simulink model "IEEE9BusSystem"  (R2024a)
settings: Solver=FixedStepAuto  StartTime=0  StopTime=100  FixedStep=Ts  RelTol=1e-3  AbsTol=1e-3  EnableMultiTasking=on
PreLoadFcn:
  | Ts = 1/60;
libraries: ee_lib x63, nesl_utility x48, fl_lib x22, eeGeneralControl x6, spsFrequencyPhasorLib x3, eeSmAC1C x3, eeSmPSS1A x3, spspowerguiLib x1
(part 2 of 2)

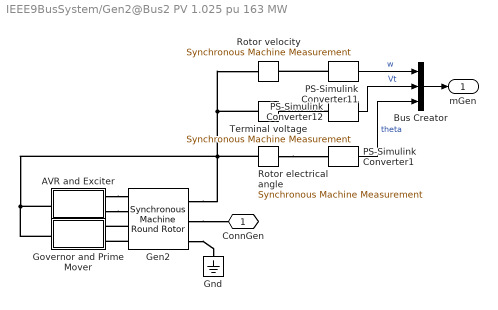
== system IEEE9BusSystem/Gen2@Bus2 PV 1.025 pu 163 MW ==
  AVR and Exciter : Subsystem
  Bus Creator : BusCreator  Inputs=3
  Gen2 : ee_lib/Electromechanical/Synchronous/Synchronous Machine Round Rotor  port_option=ee.enum.threePhasePort.composite  SRated=192 MW  VRated=18 kV  FRated=60 Hz  nPolePairs=1  param_option=ee.enum.sm.parameterization.standard  fieldCircuitParameterization_option=ee.enum.sm.fieldparameterization.current  baseEfd=92.95 V  baseIfd=100 A  zero_sequence=ee.enum.park.zerosequence.include  axes_param=ee.enum.rotorangle.qaxis  Ladu=1.6801  Laqu=1.62  L0=0.0399  Ll=0.0399  Ra=0.01  Lfd=0.2162  Rfd=8.558e-4  L1d=0.4343  R1d=0.0325  L1q=0.2635  R1q=0.0326  L2q=0.4627  R2q=0.0131  Xl=0.1  Xd=1.7199  Xq=1.6598  X0=0.1  Xdd=0.23  Xqd=0.378  Xddd=0.1728  Xqdd=0.192  d_option=ee.enum.circuit.open  Td0d=6 s  Tdd=1.3260 s  Td0dd=0.05 s  Tddd=0.0230 s  q_option=ee.enum.circuit.open  Tq0d=0.535 s  Tqd=0.3693 s  Tq0dd=0.04 s  Tqdd=0.0269 s  saturation_option=ee.enum.saturation.exclude  saturation_ifd=[0.0, 0.48, 0.76, 1.38, 1.79]  saturation_Vag=[0.0, 0.8, 1.08, 1.31, 1.4]  initialization_option=ee.enum.sm.initialization.steadystate  source_type=ee.enum.sm.load_flow_source_type.PV  Vmag0=18*1.025 kV  Vang0=0 deg  Pt0=163 MW  Qt0=0 V*A  minimum_pu=0.95  phase_search_range=[-30, 30] deg  gmin=1e-6 S  connection_option=ee.enum.Connection.wye  num_q_dampers=2  rotor_offset=-pi / 2 rad  pu_psid_specify=on  pu_psid_priority=High  pu_psid=0  pu_psid_nominal_specify=off  pu_psid_nominal_value=1  pu_psid_nominal_unit=1  pu_psiq_specify=on  pu_psiq_priority=High  pu_psiq=0  pu_psiq_nominal_specify=off  pu_psiq_nominal_value=1  pu_psiq_nominal_unit=1  pu_psifd_specify=on  pu_psifd_priority=High  pu_psifd=0  pu_psifd_nominal_specify=off  pu_psifd_nominal_value=1  pu_psifd_nominal_unit=1  pu_psi1d_specify=on  pu_psi1d_priority=High  pu_psi1d=0  pu_psi1d_nominal_specify=off  pu_psi1d_nominal_value=1  pu_psi1d_nominal_unit=1  pu_psi1q_specify=on  pu_psi1q_priority=High  pu_psi1q=0  pu_psi1q_nominal_specify=off  pu_psi1q_nominal_value=1  pu_psi1q_nominal_unit=1  pu_psi2q_specify=on  pu_psi2q_priority=High  pu_psi2q=0  pu_psi2q_nominal_specify=off  pu_psi2q_nominal_value=1  pu_psi2q_nominal_unit=1  angular_position_diff_specify=off  angular_position_diff_priority=None  angular_position_diff=0 deg  angular_position_diff_nominal_specify=off  angular_position_diff_nominal_value=1  angular_position_diff_nominal_unit=deg  Tmeas=298.15 K  alpha=3.93e-3 1/K  stator_thermal_mass=100 J/K  rotor_thermal_mass=200 J/K  temperatureA_specify=off  temperatureA_priority=High  temperatureA=25 degC  temperatureA_nominal_specify=off  temperatureA_nominal_value=1  temperatureA_nominal_unit=degC  temperatureB_specify=off  temperatureB_priority=High  temperatureB=25 degC  temperatureB_nominal_specify=off  temperatureB_nominal_value=1  temperatureB_nominal_unit=degC  temperatureC_specify=off  temperatureC_priority=High  temperatureC=25 degC  temperatureC_nominal_specify=off  temperatureC_nominal_value=1  temperatureC_nominal_unit=degC  temperatureR_specify=off  temperatureR_priority=High  temperatureR=25 degC  temperatureR_nominal_specify=off  temperatureR_nominal_value=1  temperatureR_nominal_unit=degC
      settings: InternalSimscapePortConfiguration="{\"Bottom\":[],\"Left\":[{\"id\":\"fd_p\",\"label\":\"fd+\",\"type\":\"foundation.electrical.electrical\"},{\"id\":\"fd_n\",\"label\":\"fd-\",\"type\":\"foundation.electrical.electrical\"},{\"id\":\"R\",\"label\":\"R\",\"type\":\"foundation.mechanical.rotational.rotational\"},{\"id\":\"C\",\"label\":\"C\",\"type\":\"foundation.mechanical.rotational.rotational\"}],\"Right\":[{\"id\":\"pu_output\",\"label\":\"pu\",\"type\":\"output\"},{\"id\":\"N\",\"label\":\"~\",\"type\":\"foundation.electrical.three_phase\"},{\"id\":\"n\",\"label\":\"n\",\"type\":\"foundation.electrical.electrical\"}],\"Top\":[]}"
  Gnd : fl_lib/Electrical/Electrical Elements/Electrical Reference
  Governor and Prime Mover : Subsystem
  PS-Simulink Converter1 : nesl_utility/PS-Simulink Converter  PhysicalDomain=network_engine_domain  SubClassName=ps_output  LeftPortType=input  RightPortType=output  PseudoPeriodic=off  Frequencies=[]  VectorFormat=1-D array  Unit=1  AffineConversion=off
  PS-Simulink Converter11 : nesl_utility/PS-Simulink Converter  PhysicalDomain=network_engine_domain  SubClassName=ps_output  LeftPortType=input  RightPortType=output  PseudoPeriodic=off  Frequencies=[]  VectorFormat=1-D array  Unit=1  AffineConversion=off
  PS-Simulink Converter12 : nesl_utility/PS-Simulink Converter  PhysicalDomain=network_engine_domain  SubClassName=ps_output  LeftPortType=input  RightPortType=output  PseudoPeriodic=off  Frequencies=[]  VectorFormat=1-D array  Unit=1  AffineConversion=off
  Rotor electrical angle : ee_lib/Electromechanical/Synchronous/Synchronous Machine Measurement  output_idx=19
      settings: InternalSimscapePortConfiguration="{\"Bottom\":[],\"Left\":[{\"id\":\"pu_input\",\"label\":\"pu\",\"type\":\"input\"}],\"Right\":[{\"id\":\"pu_output\",\"label\":\"o\",\"type\":\"output\"}],\"Top\":[]}"
  Rotor velocity : ee_lib/Electromechanical/Synchronous/Synchronous Machine Measurement  output_idx=4
      settings: InternalSimscapePortConfiguration="{\"Bottom\":[],\"Left\":[{\"id\":\"pu_input\",\"label\":\"pu\",\"type\":\"input\"}],\"Right\":[{\"id\":\"pu_output\",\"label\":\"o\",\"type\":\"output\"}],\"Top\":[]}"
  Terminal voltage : ee_lib/Electromechanical/Synchronous/Synchronous Machine Measurement  output_idx=14
      settings: InternalSimscapePortConfiguration="{\"Bottom\":[],\"Left\":[{\"id\":\"pu_input\",\"label\":\"pu\",\"type\":\"input\"}],\"Right\":[{\"id\":\"pu_output\",\"label\":\"o\",\"type\":\"output\"}],\"Top\":[]}"
  ConnGen : PMIOPort  Side=Right
  mGen : Outport
  wires:
  PS-Simulink Converter11/1 -> Bus Creator/1  "w"
  Bus Creator/1 -> mGen/1
  PS-Simulink Converter12/1 -> Bus Creator/2  "Vt"
  PS-Simulink Converter1/1 -> Bus Creator/3  "theta"
  connections:
  AVR and Exciter/RConn1 -- Gen2/LConn1
  AVR and Exciter/RConn2 -- Gen2/LConn2
  Gen2/LConn3 -- Governor and Prime Mover/RConn1
  Gen2/LConn4 -- Governor and Prime Mover/RConn2
  Gen2/RConn2 -- ConnGen/RConn1
  Gen2/RConn3 -- Gnd/LConn1
  Gen2/RConn1 -- AVR and Exciter/LConn1 -- Governor and Prime Mover/LConn1 -- Rotor electrical angle/LConn1 -- Rotor velocity/LConn1 -- Terminal voltage/LConn1
  PS-Simulink Converter11/LConn1 -- Rotor velocity/RConn1
  PS-Simulink Converter12/LConn1 -- Terminal voltage/RConn1
  Rotor electrical angle/RConn1 -- PS-Simulink Converter1/LConn1

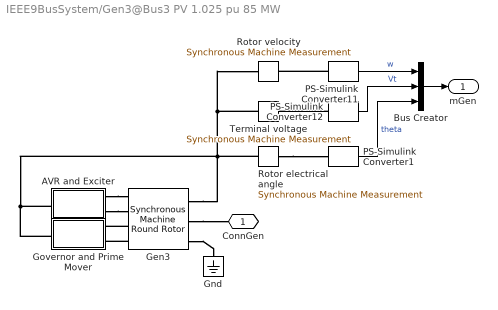
== system IEEE9BusSystem/Gen3@Bus3 PV 1.025 pu 85 MW ==
  AVR and Exciter : Subsystem
  Bus Creator : BusCreator  Inputs=3
  Gen3 : ee_lib/Electromechanical/Synchronous/Synchronous Machine Round Rotor  port_option=ee.enum.threePhasePort.composite  SRated=128 MW  VRated=13.8 kV  FRated=60 Hz  nPolePairs=1  param_option=ee.enum.sm.parameterization.standard  fieldCircuitParameterization_option=ee.enum.sm.fieldparameterization.current  baseEfd=92.95 V  baseIfd=100 A  zero_sequence=ee.enum.park.zerosequence.include  axes_param=ee.enum.rotorangle.qaxis  Ladu=1.5958  Laqu=1.5257  L0=0.0842  Ll=0.0842  Ra=0.01  Lfd=0.1715  Rfd=8.4749e-4  L1d=0.061  R1d=0.0108  L1q=0.1726  R1q=0.0222  L2q=0.3535  R2q=0.0144  Xl=0.095  Xd=1.68  Xq=1.61  X0=0.095  Xdd=0.2321  Xqd=0.32  Xddd=0.128  Xqdd=0.192  d_option=ee.enum.circuit.open  Td0d=5.89 s  Tdd=1.3260 s  Td0dd=0.05 s  Tddd=0.0230 s  q_option=ee.enum.circuit.open  Tq0d=0.6 s  Tqd=0.3693 s  Tq0dd=0.04 s  Tqdd=0.0269 s  saturation_option=ee.enum.saturation.exclude  saturation_ifd=[0.0, 0.48, 0.76, 1.38, 1.79]  saturation_Vag=[0.0, 0.8, 1.08, 1.31, 1.4]  initialization_option=ee.enum.sm.initialization.steadystate  source_type=ee.enum.sm.load_flow_source_type.PV  Vmag0=13.8*1.025 kV  Vang0=0 deg  Pt0=85 MW  Qt0=0 V*A  minimum_pu=0.95  phase_search_range=[-30, 30] deg  gmin=1e-6 S  connection_option=ee.enum.Connection.wye  num_q_dampers=2  rotor_offset=-pi / 2 rad  pu_psid_specify=on  pu_psid_priority=High  pu_psid=0  pu_psid_nominal_specify=off  pu_psid_nominal_value=1  pu_psid_nominal_unit=1  pu_psiq_specify=on  pu_psiq_priority=High  pu_psiq=0  pu_psiq_nominal_specify=off  pu_psiq_nominal_value=1  pu_psiq_nominal_unit=1  pu_psifd_specify=on  pu_psifd_priority=High  pu_psifd=0  pu_psifd_nominal_specify=off  pu_psifd_nominal_value=1  pu_psifd_nominal_unit=1  pu_psi1d_specify=on  pu_psi1d_priority=High  pu_psi1d=0  pu_psi1d_nominal_specify=off  pu_psi1d_nominal_value=1  pu_psi1d_nominal_unit=1  pu_psi1q_specify=on  pu_psi1q_priority=High  pu_psi1q=0  pu_psi1q_nominal_specify=off  pu_psi1q_nominal_value=1  pu_psi1q_nominal_unit=1  pu_psi2q_specify=on  pu_psi2q_priority=High  pu_psi2q=0  pu_psi2q_nominal_specify=off  pu_psi2q_nominal_value=1  pu_psi2q_nominal_unit=1  angular_position_diff_specify=off  angular_position_diff_priority=High  angular_position_diff=0 deg  angular_position_diff_nominal_specify=off  angular_position_diff_nominal_value=1  angular_position_diff_nominal_unit=deg  Tmeas=298.15 K  alpha=3.93e-3 1/K  stator_thermal_mass=100 J/K  rotor_thermal_mass=200 J/K  temperatureA_specify=off  temperatureA_priority=High  temperatureA=25 degC  temperatureA_nominal_specify=off  temperatureA_nominal_value=1  temperatureA_nominal_unit=degC  temperatureB_specify=off  temperatureB_priority=High  temperatureB=25 degC  temperatureB_nominal_specify=off  temperatureB_nominal_value=1  temperatureB_nominal_unit=degC  temperatureC_specify=off  temperatureC_priority=High  temperatureC=25 degC  temperatureC_nominal_specify=off  temperatureC_nominal_value=1  temperatureC_nominal_unit=degC  temperatureR_specify=off  temperatureR_priority=High  temperatureR=25 degC  temperatureR_nominal_specify=off  temperatureR_nominal_value=1  temperatureR_nominal_unit=degC
      settings: InternalSimscapePortConfiguration="{\"Bottom\":[],\"Left\":[{\"id\":\"fd_p\",\"label\":\"fd+\",\"type\":\"foundation.electrical.electrical\"},{\"id\":\"fd_n\",\"label\":\"fd-\",\"type\":\"foundation.electrical.electrical\"},{\"id\":\"R\",\"label\":\"R\",\"type\":\"foundation.mechanical.rotational.rotational\"},{\"id\":\"C\",\"label\":\"C\",\"type\":\"foundation.mechanical.rotational.rotational\"}],\"Right\":[{\"id\":\"pu_output\",\"label\":\"pu\",\"type\":\"output\"},{\"id\":\"N\",\"label\":\"~\",\"type\":\"foundation.electrical.three_phase\"},{\"id\":\"n\",\"label\":\"n\",\"type\":\"foundation.electrical.electrical\"}],\"Top\":[]}"
  Gnd : fl_lib/Electrical/Electrical Elements/Electrical Reference
  Governor and Prime Mover : Subsystem
  PS-Simulink Converter1 : nesl_utility/PS-Simulink Converter  PhysicalDomain=network_engine_domain  SubClassName=ps_output  LeftPortType=input  RightPortType=output  PseudoPeriodic=off  Frequencies=[]  VectorFormat=1-D array  Unit=1  AffineConversion=off
  PS-Simulink Converter11 : nesl_utility/PS-Simulink Converter  PhysicalDomain=network_engine_domain  SubClassName=ps_output  LeftPortType=input  RightPortType=output  PseudoPeriodic=off  Frequencies=[]  VectorFormat=1-D array  Unit=1  AffineConversion=off
  PS-Simulink Converter12 : nesl_utility/PS-Simulink Converter  PhysicalDomain=network_engine_domain  SubClassName=ps_output  LeftPortType=input  RightPortType=output  PseudoPeriodic=off  Frequencies=[]  VectorFormat=1-D array  Unit=1  AffineConversion=off
  Rotor electrical angle : ee_lib/Electromechanical/Synchronous/Synchronous Machine Measurement  output_idx=19
      settings: InternalSimscapePortConfiguration="{\"Bottom\":[],\"Left\":[{\"id\":\"pu_input\",\"label\":\"pu\",\"type\":\"input\"}],\"Right\":[{\"id\":\"pu_output\",\"label\":\"o\",\"type\":\"output\"}],\"Top\":[]}"
  Rotor velocity : ee_lib/Electromechanical/Synchronous/Synchronous Machine Measurement  output_idx=4
      settings: InternalSimscapePortConfiguration="{\"Bottom\":[],\"Left\":[{\"id\":\"pu_input\",\"label\":\"pu\",\"type\":\"input\"}],\"Right\":[{\"id\":\"pu_output\",\"label\":\"o\",\"type\":\"output\"}],\"Top\":[]}"
  Terminal voltage : ee_lib/Electromechanical/Synchronous/Synchronous Machine Measurement  output_idx=14
      settings: InternalSimscapePortConfiguration="{\"Bottom\":[],\"Left\":[{\"id\":\"pu_input\",\"label\":\"pu\",\"type\":\"input\"}],\"Right\":[{\"id\":\"pu_output\",\"label\":\"o\",\"type\":\"output\"}],\"Top\":[]}"
  ConnGen : PMIOPort  Side=Right
  mGen : Outport
  wires:
  PS-Simulink Converter1/1 -> Bus Creator/3  "theta"
  PS-Simulink Converter12/1 -> Bus Creator/2  "Vt"
  Bus Creator/1 -> mGen/1
  PS-Simulink Converter11/1 -> Bus Creator/1  "w"
  connections:
  Rotor electrical angle/RConn1 -- PS-Simulink Converter1/LConn1
  PS-Simulink Converter12/LConn1 -- Terminal voltage/RConn1
  PS-Simulink Converter11/LConn1 -- Rotor velocity/RConn1
  Terminal voltage/LConn1 -- Gen3/RConn1 -- Rotor electrical angle/LConn1 -- AVR and Exciter/LConn1 -- Governor and Prime Mover/LConn1 -- Rotor velocity/LConn1
  Gen3/RConn3 -- Gnd/LConn1
  Gen3/RConn2 -- ConnGen/RConn1
  Gen3/LConn4 -- Governor and Prime Mover/RConn2
  Gen3/LConn3 -- Governor and Prime Mover/RConn1
  AVR and Exciter/RConn2 -- Gen3/LConn2
  AVR and Exciter/RConn1 -- Gen3/LConn1

== system IEEE9BusSystem/Scope ==
  BusElementIn : Inport  PortName=mGen1  Element=w
  BusElementIn1 : Inport  PortName=mGen1  Element=Vt
  BusElementIn2 : Inport  Port=2  PortName=mGen2  Element=Vt
  BusElementIn4 : Inport  Port=2  PortName=mGen2  Element=w
  BusElementIn3 : Inport  Port=3  PortName=mGen3  Element=Vt
  BusElementIn5 : Inport  Port=3  PortName=mGen3  Element=w
  Mux : Mux  Inputs=3
  Mux1 : Mux  Inputs=3
  Scope : Scope  NumInputPorts=2
  wires:
  BusElementIn4/1 -> Mux/2
  BusElementIn/1 -> Mux/1
  BusElementIn5/1 -> Mux/3
  BusElementIn1/1 -> Mux1/1
  BusElementIn2/1 -> Mux1/2
  BusElementIn3/1 -> Mux1/3
  Mux1/1 -> Scope/1  "Terminal voltages [p.u.]"
  Mux/1 -> Scope/2  "Rotor speeds [p.u.]"

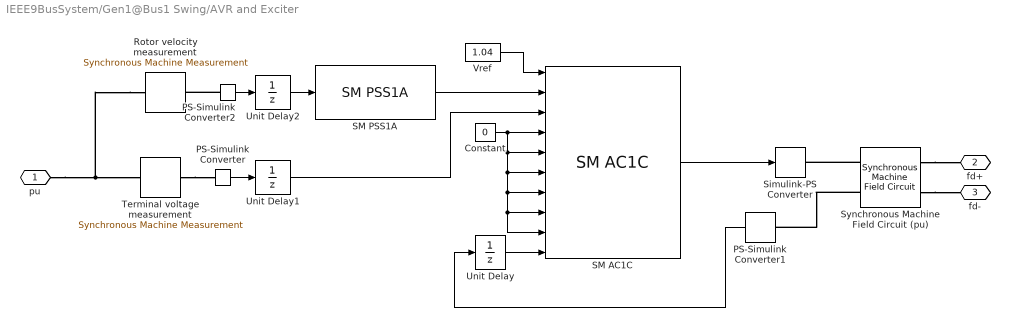
== system IEEE9BusSystem/Gen1@Bus1 Swing/AVR and Exciter ==
  Constant : Constant  Value=0
  PS-Simulink Converter : nesl_utility/PS-Simulink Converter  PhysicalDomain=network_engine_domain  SubClassName=ps_output  LeftPortType=input  RightPortType=output  PseudoPeriodic=off  Frequencies=[]  VectorFormat=1-D array  Unit=1  AffineConversion=off
  PS-Simulink Converter1 : nesl_utility/PS-Simulink Converter  PhysicalDomain=network_engine_domain  SubClassName=ps_output  LeftPortType=input  RightPortType=output  PseudoPeriodic=off  Frequencies=[]  VectorFormat=1-D array  Unit=1  AffineConversion=off
  PS-Simulink Converter2 : nesl_utility/PS-Simulink Converter  PhysicalDomain=network_engine_domain  SubClassName=ps_output  LeftPortType=input  RightPortType=output  PseudoPeriodic=off  Frequencies=[]  VectorFormat=1-D array  Unit=1  AffineConversion=off
  Rotor velocity measurement : ee_lib/Electromechanical/Synchronous/Synchronous Machine Measurement  output_idx=4
      settings: InternalSimscapePortConfiguration="{\"Bottom\":[],\"Left\":[{\"id\":\"pu_input\",\"label\":\"pu\",\"type\":\"input\"}],\"Right\":[{\"id\":\"pu_output\",\"label\":\"o\",\"type\":\"output\"}],\"Top\":[]}"
  SM AC1C : eeSmAC1C/SM AC1C  E_FD0=1.08614  Ts=Ts  R_C=0  X_C=0  T_R=0  K_A=400  T_A=0.02  T_B=0  T_C=0  K_F=0.03  T_F=1  V_Amax=14.5  V_Amin=-14.5  E_FEmax=6.03  E_FEmin=-5.43  oelInputLocation=Unused  uelInputLocation=Unused  sclInputLocation=Unused  K_E=1  T_E=0.8  K_C=0.2  K_D=0.38  E_1=4.18  S_E_E1=0.1  E_2=3.14  S_E_E2=0.03  V_FEmax=99  V_Emin=0
  SM PSS1A : eeSmPSS1A/SM PSS1A  K_S=3.15  A_1=0  A_2=0  T_1=0  T_2=0  T_3=0.32  T_4=0.016  T_5=1  T_6=0.0106  V_STmax=0.09  V_STmin=-0.09  Ts=Ts
  Simulink-PS Converter : nesl_utility/Simulink-PS Converter  PhysicalDomain=network_engine_domain  SubClassName=ps_input  LeftPortType=input  RightPortType=output  PseudoPeriodic=off  Frequencies=[]  NoiseDistribution=none  NoiseParameters=[]  Unit=1  AffineConversion=off  FilteringAndDerivatives=provide  SimscapeFilterOrder=1  InputFilterTimeConstant=0.001  UdotUserProvided=0
  Synchronous Machine Field Circuit (pu) : ee_lib/Electromechanical/Synchronous/Synchronous Machine Field Circuit  unit_option=ee.enum.unit.pu  SRated=247.5 MW  FRated=60 Hz  fieldCircuitParameterization_option=ee.enum.sm.fieldparameterization.current  baseEfd=92.95 V  baseIfd=100 A  parameterization_option=ee.enum.sm.parameterization.standard  Ladu=0.2725  Rfd=1.0656e-4  Xl=0.0832  Xd=0.3614  Xdd=0.1505  Xddd=0.0990  d_option=ee.enum.circuit.open  Td0d=8.96 s  Tdd=1.3260 s  Td0dd=0.05 s  Tddd=0.0230 s
      settings: InternalSimscapePortConfiguration="{\"Bottom\":[],\"Left\":[{\"id\":\"Efd_pu\",\"label\":\"Efd_pu\",\"type\":\"input\"},{\"id\":\"Ifd_pu\",\"label\":\"Ifd_pu\",\"type\":\"output\"}],\"Right\":[{\"id\":\"fd_p\",\"label\":\"fd+\",\"type\":\"foundation.electrical.electrical\"},{\"id\":\"fd_n\",\"label\":\"fd-\",\"type\":\"foundation.electrical.electrical\"}],\"Top\":[]}"
  Terminal voltage measurement : ee_lib/Electromechanical/Synchronous/Synchronous Machine Measurement  output_idx=14
      settings: InternalSimscapePortConfiguration="{\"Bottom\":[],\"Left\":[{\"id\":\"pu_input\",\"label\":\"pu\",\"type\":\"input\"}],\"Right\":[{\"id\":\"pu_output\",\"label\":\"o\",\"type\":\"output\"}],\"Top\":[]}"
  Unit Delay : UnitDelay  InitialCondition=1.08614  SampleTime=Ts  HasFrameUpgradeWarning=on
  Unit Delay1 : UnitDelay  InitialCondition=1.04  SampleTime=Ts  HasFrameUpgradeWarning=on
  Unit Delay2 : UnitDelay  InitialCondition=1  SampleTime=Ts  HasFrameUpgradeWarning=on
  Vref : Constant  Value=1.04
  pu : PMIOPort  Side=Left
  fd+ : PMIOPort  Port=2  Side=Right
  fd- : PMIOPort  Port=3  Side=Right
  wires:
  Unit Delay2/1 -> SM PSS1A/1
  PS-Simulink Converter2/1 -> Unit Delay2/1
  Unit Delay1/1 -> SM AC1C/3
  Vref/1 -> SM AC1C/1
  Constant/1 -> SM AC1C/9, SM AC1C/8, SM AC1C/7, SM AC1C/6, SM AC1C/5, SM AC1C/4
  Unit Delay/1 -> SM AC1C/10
  SM AC1C/1 -> Simulink-PS Converter/1
  PS-Simulink Converter1/1 -> Unit Delay/1
  SM PSS1A/1 -> SM AC1C/2
  PS-Simulink Converter/1 -> Unit Delay1/1
  connections:
  PS-Simulink Converter2/LConn1 -- Rotor velocity measurement/RConn1
  Rotor velocity measurement/LConn1 -- Terminal voltage measurement/LConn1 -- pu/RConn1
  Terminal voltage measurement/RConn1 -- PS-Simulink Converter/LConn1
  Synchronous Machine Field Circuit (pu)/LConn1 -- Simulink-PS Converter/RConn1
  Synchronous Machine Field Circuit (pu)/LConn2 -- PS-Simulink Converter1/LConn1
  Synchronous Machine Field Circuit (pu)/RConn2 -- fd-/RConn1
  Synchronous Machine Field Circuit (pu)/RConn1 -- fd+/RConn1

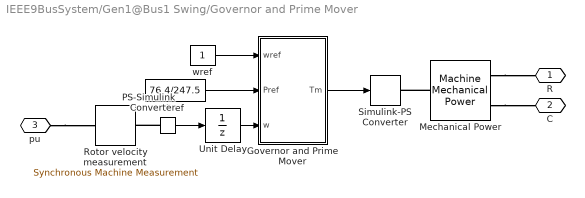
== system IEEE9BusSystem/Gen1@Bus1 Swing/Governor and Prime Mover ==
  "Governor and Prime Mover " : Subsystem  mask(Governor and Prime Mover){droop_percentage=5, Tg=0.15, Tch=0.3, pu_torque0=0.309487, Ts=Ts}
      mask prompts: droop_percentage "Percentage droop, (%)"; Tg "Time constant of governor, Tg (s)"; Tch "Time constant of main inlet volumes and steam chest, Tch (s)"; pu_torque0 "Initial torque, (pu)"; Ts "Sample time"
      mask help:
      | Implements a synchronous machine governor and prime mover. The prime mover is a non-reheat steam turbine.
      |
      | The input to the block is a per-unit synchronous machine measurement vector.
      |
      | R and C are mechanical rotational ports.
  Mechanical Power : ee_lib/Electromechanical/Mechanical/Machine Mechanical Power  power_sign=-1  SRated=247.5 MW  FRated=60 Hz  nPolePairs=20  inputUnit=ee.enum.unit.pu  torque_factor=2  inertia_option=2  J=27548 kg*m^2  H=9.5515 W*s/(A*V)  damper_option=2  D=39.0509 N*m*s/rad  pu_D=0  initialization_option=2  fMechanical0=60 Hz  fElectrical0=60 Hz
      settings: InternalSimscapePortConfiguration="{\"Bottom\":[],\"Left\":[{\"id\":\"Pm_pu\",\"label\":\"pu\",\"type\":\"input\"}],\"Right\":[{\"id\":\"R\",\"label\":\"R\",\"type\":\"foundation.mechanical.rotational.rotational\"},{\"id\":\"C\",\"label\":\"C\",\"type\":\"foundation.mechanical.rotational.rotational\"}],\"Top\":[]}"
  PS-Simulink Converter : nesl_utility/PS-Simulink Converter  PhysicalDomain=network_engine_domain  SubClassName=ps_output  LeftPortType=input  RightPortType=output  PseudoPeriodic=off  Frequencies=[]  VectorFormat=1-D array  Unit=1  AffineConversion=off
  Pref : Constant  Value=76.4/247.5
  Rotor velocity measurement : ee_lib/Electromechanical/Synchronous/Synchronous Machine Measurement  output_idx=4
      settings: InternalSimscapePortConfiguration="{\"Bottom\":[],\"Left\":[{\"id\":\"pu_input\",\"label\":\"pu\",\"type\":\"input\"}],\"Right\":[{\"id\":\"pu_output\",\"label\":\"o\",\"type\":\"output\"}],\"Top\":[]}"
  Simulink-PS Converter : nesl_utility/Simulink-PS Converter  PhysicalDomain=network_engine_domain  SubClassName=ps_input  LeftPortType=input  RightPortType=output  PseudoPeriodic=off  Frequencies=[]  NoiseDistribution=none  NoiseParameters=[]  Unit=1  AffineConversion=off  FilteringAndDerivatives=provide  SimscapeFilterOrder=1  InputFilterTimeConstant=0.001  UdotUserProvided=0
  Unit Delay : UnitDelay  InitialCondition=1  SampleTime=Ts  HasFrameUpgradeWarning=on
  wref : Constant
  R : PMIOPort  Side=Right
  C : PMIOPort  Port=2  Side=Right
  pu : PMIOPort  Port=3  Side=Left
  wires:
  PS-Simulink Converter/1 -> Unit Delay/1
  Unit Delay/1 -> "Governor and Prime Mover "/3(w)
  Pref/1 -> "Governor and Prime Mover "/2(Pref)
  "Governor and Prime Mover "/1(Tm) -> Simulink-PS Converter/1
  wref/1 -> "Governor and Prime Mover "/1(wref)
  connections:
  PS-Simulink Converter/LConn1 -- Rotor velocity measurement/RConn1
  Mechanical Power/RConn1 -- R/RConn1
  pu/RConn1 -- Rotor velocity measurement/LConn1
  Mechanical Power/RConn2 -- C/RConn1
  Mechanical Power/LConn1 -- Simulink-PS Converter/RConn1

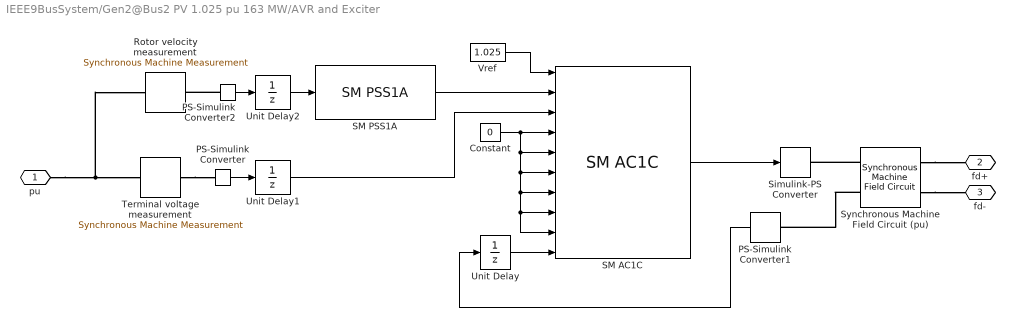
== system IEEE9BusSystem/Gen2@Bus2 PV 1.025 pu 163 MW/AVR and Exciter ==
  Constant : Constant  Value=0
  PS-Simulink Converter : nesl_utility/PS-Simulink Converter  PhysicalDomain=network_engine_domain  SubClassName=ps_output  LeftPortType=input  RightPortType=output  PseudoPeriodic=off  Frequencies=[]  VectorFormat=1-D array  Unit=1  AffineConversion=off
  PS-Simulink Converter1 : nesl_utility/PS-Simulink Converter  PhysicalDomain=network_engine_domain  SubClassName=ps_output  LeftPortType=input  RightPortType=output  PseudoPeriodic=off  Frequencies=[]  VectorFormat=1-D array  Unit=1  AffineConversion=off
  PS-Simulink Converter2 : nesl_utility/PS-Simulink Converter  PhysicalDomain=network_engine_domain  SubClassName=ps_output  LeftPortType=input  RightPortType=output  PseudoPeriodic=off  Frequencies=[]  VectorFormat=1-D array  Unit=1  AffineConversion=off
  Rotor velocity measurement : ee_lib/Electromechanical/Synchronous/Synchronous Machine Measurement  output_idx=4
      settings: InternalSimscapePortConfiguration="{\"Bottom\":[],\"Left\":[{\"id\":\"pu_input\",\"label\":\"pu\",\"type\":\"input\"}],\"Right\":[{\"id\":\"pu_output\",\"label\":\"o\",\"type\":\"output\"}],\"Top\":[]}"
  SM AC1C : eeSmAC1C/SM AC1C  E_FD0=1.79759  Ts=Ts  R_C=0  X_C=0  T_R=0  K_A=400  T_A=0.02  T_B=0  T_C=0  K_F=0.03  T_F=1  V_Amax=14.5  V_Amin=-14.5  E_FEmax=6.03  E_FEmin=-5.43  oelInputLocation=Unused  uelInputLocation=Unused  sclInputLocation=Unused  K_E=1  T_E=0.8  K_C=0.2  K_D=0.38  E_1=4.18  S_E_E1=0.1  E_2=3.14  S_E_E2=0.03  V_FEmax=99  V_Emin=0
  SM PSS1A : eeSmPSS1A/SM PSS1A  K_S=3.15  A_1=0  A_2=0  T_1=0  T_2=0  T_3=0.32  T_4=0.016  T_5=1  T_6=0.0106  V_STmax=0.09  V_STmin=-0.09  Ts=Ts
  Simulink-PS Converter : nesl_utility/Simulink-PS Converter  PhysicalDomain=network_engine_domain  SubClassName=ps_input  LeftPortType=input  RightPortType=output  PseudoPeriodic=off  Frequencies=[]  NoiseDistribution=none  NoiseParameters=[]  Unit=1  AffineConversion=off  FilteringAndDerivatives=provide  SimscapeFilterOrder=1  InputFilterTimeConstant=0.001  UdotUserProvided=0
  Synchronous Machine Field Circuit (pu) : ee_lib/Electromechanical/Synchronous/Synchronous Machine Field Circuit  unit_option=ee.enum.unit.pu  SRated=192 MW  FRated=60 Hz  fieldCircuitParameterization_option=ee.enum.sm.fieldparameterization.current  baseEfd=92.95 V  baseIfd=100 A  parameterization_option=ee.enum.sm.parameterization.standard  Ladu=1.6801  Rfd=8.558e-4  Xl=0.1  Xd=1.7199  Xdd=0.23  Xddd=0.1728  d_option=ee.enum.circuit.open  Td0d=6 s  Tdd=1.3260 s  Td0dd=0.05 s  Tddd=0.0230 s
      settings: InternalSimscapePortConfiguration="{\"Bottom\":[],\"Left\":[{\"id\":\"Efd_pu\",\"label\":\"Efd_pu\",\"type\":\"input\"},{\"id\":\"Ifd_pu\",\"label\":\"Ifd_pu\",\"type\":\"output\"}],\"Right\":[{\"id\":\"fd_p\",\"label\":\"fd+\",\"type\":\"foundation.electrical.electrical\"},{\"id\":\"fd_n\",\"label\":\"fd-\",\"type\":\"foundation.electrical.electrical\"}],\"Top\":[]}"
  Terminal voltage measurement : ee_lib/Electromechanical/Synchronous/Synchronous Machine Measurement  output_idx=14
      settings: InternalSimscapePortConfiguration="{\"Bottom\":[],\"Left\":[{\"id\":\"pu_input\",\"label\":\"pu\",\"type\":\"input\"}],\"Right\":[{\"id\":\"pu_output\",\"label\":\"o\",\"type\":\"output\"}],\"Top\":[]}"
  Unit Delay : UnitDelay  InitialCondition=1.79759  SampleTime=Ts  HasFrameUpgradeWarning=on
  Unit Delay1 : UnitDelay  InitialCondition=1.025  SampleTime=Ts  HasFrameUpgradeWarning=on
  Unit Delay2 : UnitDelay  InitialCondition=1  SampleTime=Ts  HasFrameUpgradeWarning=on
  Vref : Constant  Value=1.025
  pu : PMIOPort  Side=Left
  fd+ : PMIOPort  Port=2  Side=Right
  fd- : PMIOPort  Port=3  Side=Right
  wires:
  PS-Simulink Converter/1 -> Unit Delay1/1
  SM PSS1A/1 -> SM AC1C/2
  PS-Simulink Converter1/1 -> Unit Delay/1
  SM AC1C/1 -> Simulink-PS Converter/1
  Unit Delay/1 -> SM AC1C/10
  Constant/1 -> SM AC1C/4, SM AC1C/5, SM AC1C/6, SM AC1C/7, SM AC1C/8, SM AC1C/9
  Vref/1 -> SM AC1C/1
  Unit Delay1/1 -> SM AC1C/3
  Unit Delay2/1 -> SM PSS1A/1
  PS-Simulink Converter2/1 -> Unit Delay2/1
  connections:
  Synchronous Machine Field Circuit (pu)/RConn1 -- fd+/RConn1
  Synchronous Machine Field Circuit (pu)/RConn2 -- fd-/RConn1
  Synchronous Machine Field Circuit (pu)/LConn2 -- PS-Simulink Converter1/LConn1
  Synchronous Machine Field Circuit (pu)/LConn1 -- Simulink-PS Converter/RConn1
  Terminal voltage measurement/RConn1 -- PS-Simulink Converter/LConn1
  pu/RConn1 -- Terminal voltage measurement/LConn1 -- Rotor velocity measurement/LConn1
  PS-Simulink Converter2/LConn1 -- Rotor velocity measurement/RConn1

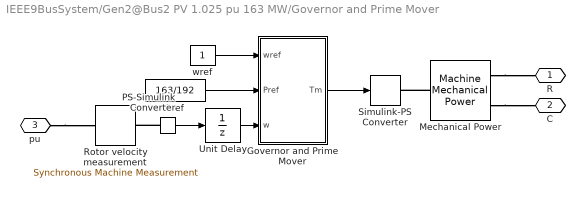
== system IEEE9BusSystem/Gen2@Bus2 PV 1.025 pu 163 MW/Governor and Prime Mover ==
  "Governor and Prime Mover " : Subsystem  mask(Governor and Prime Mover){droop_percentage=5, Tg=0.15, Tch=0.3, pu_torque0=0.855832, Ts=Ts}
      mask prompts: droop_percentage "Percentage droop, (%)"; Tg "Time constant of governor, Tg (s)"; Tch "Time constant of main inlet volumes and steam chest, Tch (s)"; pu_torque0 "Initial torque, (pu)"; Ts "Sample time"
      mask help:
      | Implements a synchronous machine governor and prime mover. The prime mover is a non-reheat steam turbine.
      |
      | The input to the block is a per-unit synchronous machine measurement vector.
      |
      | R and C are mechanical rotational ports.
  Mechanical Power : ee_lib/Electromechanical/Mechanical/Machine Mechanical Power  power_sign=-1  SRated=192 MW  FRated=60 Hz  nPolePairs=1  inputUnit=ee.enum.unit.pu  torque_factor=2  inertia_option=2  J=27548 kg*m^2  H=3.3333 W*s/(A*V)  damper_option=2  D=39.0509 N*m*s/rad  pu_D=0  initialization_option=2  fMechanical0=60 Hz  fElectrical0=60 Hz
      settings: InternalSimscapePortConfiguration="{\"Bottom\":[],\"Left\":[{\"id\":\"Pm_pu\",\"label\":\"pu\",\"type\":\"input\"}],\"Right\":[{\"id\":\"R\",\"label\":\"R\",\"type\":\"foundation.mechanical.rotational.rotational\"},{\"id\":\"C\",\"label\":\"C\",\"type\":\"foundation.mechanical.rotational.rotational\"}],\"Top\":[]}"
  PS-Simulink Converter : nesl_utility/PS-Simulink Converter  PhysicalDomain=network_engine_domain  SubClassName=ps_output  LeftPortType=input  RightPortType=output  PseudoPeriodic=off  Frequencies=[]  VectorFormat=1-D array  Unit=1  AffineConversion=off
  Pref : Constant  Value=163/192
  Rotor velocity measurement : ee_lib/Electromechanical/Synchronous/Synchronous Machine Measurement  output_idx=4
      settings: InternalSimscapePortConfiguration="{\"Bottom\":[],\"Left\":[{\"id\":\"pu_input\",\"label\":\"pu\",\"type\":\"input\"}],\"Right\":[{\"id\":\"pu_output\",\"label\":\"o\",\"type\":\"output\"}],\"Top\":[]}"
  Simulink-PS Converter : nesl_utility/Simulink-PS Converter  PhysicalDomain=network_engine_domain  SubClassName=ps_input  LeftPortType=input  RightPortType=output  PseudoPeriodic=off  Frequencies=[]  NoiseDistribution=none  NoiseParameters=[]  Unit=1  AffineConversion=off  FilteringAndDerivatives=provide  SimscapeFilterOrder=1  InputFilterTimeConstant=0.001  UdotUserProvided=0
  Unit Delay : UnitDelay  InitialCondition=1  SampleTime=Ts  HasFrameUpgradeWarning=on
  wref : Constant
  R : PMIOPort  Side=Right
  C : PMIOPort  Port=2  Side=Right
  pu : PMIOPort  Port=3  Side=Left
  wires:
  wref/1 -> "Governor and Prime Mover "/1(wref)
  "Governor and Prime Mover "/1(Tm) -> Simulink-PS Converter/1
  Pref/1 -> "Governor and Prime Mover "/2(Pref)
  Unit Delay/1 -> "Governor and Prime Mover "/3(w)
  PS-Simulink Converter/1 -> Unit Delay/1
  connections:
  Mechanical Power/LConn1 -- Simulink-PS Converter/RConn1
  Mechanical Power/RConn2 -- C/RConn1
  pu/RConn1 -- Rotor velocity measurement/LConn1
  Mechanical Power/RConn1 -- R/RConn1
  PS-Simulink Converter/LConn1 -- Rotor velocity measurement/RConn1

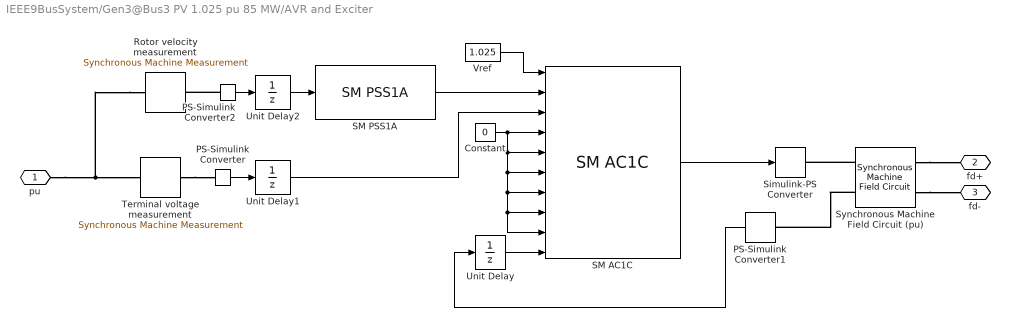
== system IEEE9BusSystem/Gen3@Bus3 PV 1.025 pu 85 MW/AVR and Exciter ==
  Constant : Constant  Value=0
  PS-Simulink Converter : nesl_utility/PS-Simulink Converter  PhysicalDomain=network_engine_domain  SubClassName=ps_output  LeftPortType=input  RightPortType=output  PseudoPeriodic=off  Frequencies=[]  VectorFormat=1-D array  Unit=1  AffineConversion=off
  PS-Simulink Converter1 : nesl_utility/PS-Simulink Converter  PhysicalDomain=network_engine_domain  SubClassName=ps_output  LeftPortType=input  RightPortType=output  PseudoPeriodic=off  Frequencies=[]  VectorFormat=1-D array  Unit=1  AffineConversion=off
  PS-Simulink Converter2 : nesl_utility/PS-Simulink Converter  PhysicalDomain=network_engine_domain  SubClassName=ps_output  LeftPortType=input  RightPortType=output  PseudoPeriodic=off  Frequencies=[]  VectorFormat=1-D array  Unit=1  AffineConversion=off
  Rotor velocity measurement : ee_lib/Electromechanical/Synchronous/Synchronous Machine Measurement  output_idx=4
      settings: InternalSimscapePortConfiguration="{\"Bottom\":[],\"Left\":[{\"id\":\"pu_input\",\"label\":\"pu\",\"type\":\"input\"}],\"Right\":[{\"id\":\"pu_output\",\"label\":\"o\",\"type\":\"output\"}],\"Top\":[]}"
  SM AC1C : eeSmAC1C/SM AC1C  E_FD0=1.41658  Ts=Ts  R_C=0  X_C=0  T_R=0  K_A=400  T_A=0.02  T_B=0  T_C=0  K_F=0.03  T_F=1  V_Amax=14.5  V_Amin=-14.5  E_FEmax=6.03  E_FEmin=-5.43  oelInputLocation=Unused  uelInputLocation=Unused  sclInputLocation=Unused  K_E=1  T_E=0.8  K_C=0.2  K_D=0.38  E_1=4.18  S_E_E1=0.1  E_2=3.14  S_E_E2=0.03  V_FEmax=99  V_Emin=0
  SM PSS1A : eeSmPSS1A/SM PSS1A  K_S=3.15  A_1=0  A_2=0  T_1=0  T_2=0  T_3=0.32  T_4=0.016  T_5=1  T_6=0.0106  V_STmax=0.09  V_STmin=-0.09  Ts=Ts
  Simulink-PS Converter : nesl_utility/Simulink-PS Converter  PhysicalDomain=network_engine_domain  SubClassName=ps_input  LeftPortType=input  RightPortType=output  PseudoPeriodic=off  Frequencies=[]  NoiseDistribution=none  NoiseParameters=[]  Unit=1  AffineConversion=off  FilteringAndDerivatives=provide  SimscapeFilterOrder=1  InputFilterTimeConstant=0.001  UdotUserProvided=0
  Synchronous Machine Field Circuit (pu) : ee_lib/Electromechanical/Synchronous/Synchronous Machine Field Circuit  unit_option=ee.enum.unit.pu  SRated=128 MW  FRated=60 Hz  fieldCircuitParameterization_option=ee.enum.sm.fieldparameterization.current  baseEfd=92.95 V  baseIfd=100 A  parameterization_option=ee.enum.sm.parameterization.standard  Ladu=1.5958  Rfd=8.4749e-4  Xl=0.095  Xd=1.68  Xdd=0.2321  Xddd=0.128  d_option=ee.enum.circuit.open  Td0d=5.89 s  Tdd=1.3260 s  Td0dd=0.05 s  Tddd=0.0230 s
      settings: InternalSimscapePortConfiguration="{\"Bottom\":[],\"Left\":[{\"id\":\"Efd_pu\",\"label\":\"Efd_pu\",\"type\":\"input\"},{\"id\":\"Ifd_pu\",\"label\":\"Ifd_pu\",\"type\":\"output\"}],\"Right\":[{\"id\":\"fd_p\",\"label\":\"fd+\",\"type\":\"foundation.electrical.electrical\"},{\"id\":\"fd_n\",\"label\":\"fd-\",\"type\":\"foundation.electrical.electrical\"}],\"Top\":[]}"
  Terminal voltage measurement : ee_lib/Electromechanical/Synchronous/Synchronous Machine Measurement  output_idx=14
      settings: InternalSimscapePortConfiguration="{\"Bottom\":[],\"Left\":[{\"id\":\"pu_input\",\"label\":\"pu\",\"type\":\"input\"}],\"Right\":[{\"id\":\"pu_output\",\"label\":\"o\",\"type\":\"output\"}],\"Top\":[]}"
  Unit Delay : UnitDelay  InitialCondition=1.41658  SampleTime=Ts  HasFrameUpgradeWarning=on
  Unit Delay1 : UnitDelay  InitialCondition=1.025  SampleTime=Ts  HasFrameUpgradeWarning=on
  Unit Delay2 : UnitDelay  InitialCondition=1  SampleTime=Ts  HasFrameUpgradeWarning=on
  Vref : Constant  Value=1.025
  pu : PMIOPort  Side=Left
  fd+ : PMIOPort  Port=2  Side=Right
  fd- : PMIOPort  Port=3  Side=Right
  wires:
  Unit Delay2/1 -> SM PSS1A/1
  PS-Simulink Converter2/1 -> Unit Delay2/1
  Unit Delay1/1 -> SM AC1C/3
  Vref/1 -> SM AC1C/1
  Constant/1 -> SM AC1C/9, SM AC1C/8, SM AC1C/7, SM AC1C/6, SM AC1C/5, SM AC1C/4
  Unit Delay/1 -> SM AC1C/10
  SM AC1C/1 -> Simulink-PS Converter/1
  PS-Simulink Converter1/1 -> Unit Delay/1
  SM PSS1A/1 -> SM AC1C/2
  PS-Simulink Converter/1 -> Unit Delay1/1
  connections:
  PS-Simulink Converter2/LConn1 -- Rotor velocity measurement/RConn1
  Rotor velocity measurement/LConn1 -- Terminal voltage measurement/LConn1 -- pu/RConn1
  Terminal voltage measurement/RConn1 -- PS-Simulink Converter/LConn1
  Synchronous Machine Field Circuit (pu)/LConn1 -- Simulink-PS Converter/RConn1
  Synchronous Machine Field Circuit (pu)/LConn2 -- PS-Simulink Converter1/LConn1
  Synchronous Machine Field Circuit (pu)/RConn2 -- fd-/RConn1
  Synchronous Machine Field Circuit (pu)/RConn1 -- fd+/RConn1

== system IEEE9BusSystem/Gen3@Bus3 PV 1.025 pu 85 MW/Governor and Prime Mover ==
  "Governor and Prime Mover " : Subsystem  mask(Governor and Prime Mover){droop_percentage=5, Tg=0.15, Tch=0.3, pu_torque0=0.668315, Ts=Ts}
      mask prompts: droop_percentage "Percentage droop, (%)"; Tg "Time constant of governor, Tg (s)"; Tch "Time constant of main inlet volumes and steam chest, Tch (s)"; pu_torque0 "Initial torque, (pu)"; Ts "Sample time"
      mask help:
      | Implements a synchronous machine governor and prime mover. The prime mover is a non-reheat steam turbine.
      |
      | The input to the block is a per-unit synchronous machine measurement vector.
      |
      | R and C are mechanical rotational ports.
  Mechanical Power : ee_lib/Electromechanical/Mechanical/Machine Mechanical Power  power_sign=-1  SRated=128 MW  FRated=60 Hz  nPolePairs=1  inputUnit=ee.enum.unit.pu  torque_factor=2  inertia_option=2  J=27548 kg*m^2  H=2.3516 W*s/(A*V)  damper_option=2  D=39.0509 N*m*s/rad  pu_D=0  initialization_option=2  fMechanical0=60 Hz  fElectrical0=60 Hz
      settings: InternalSimscapePortConfiguration="{\"Bottom\":[],\"Left\":[{\"id\":\"Pm_pu\",\"label\":\"pu\",\"type\":\"input\"}],\"Right\":[{\"id\":\"R\",\"label\":\"R\",\"type\":\"foundation.mechanical.rotational.rotational\"},{\"id\":\"C\",\"label\":\"C\",\"type\":\"foundation.mechanical.rotational.rotational\"}],\"Top\":[]}"
  PS-Simulink Converter : nesl_utility/PS-Simulink Converter  PhysicalDomain=network_engine_domain  SubClassName=ps_output  LeftPortType=input  RightPortType=output  PseudoPeriodic=off  Frequencies=[]  VectorFormat=1-D array  Unit=1  AffineConversion=off
  Pref : Constant  Value=85/128
  Rotor velocity measurement : ee_lib/Electromechanical/Synchronous/Synchronous Machine Measurement  output_idx=4
      settings: InternalSimscapePortConfiguration="{\"Bottom\":[],\"Left\":[{\"id\":\"pu_input\",\"label\":\"pu\",\"type\":\"input\"}],\"Right\":[{\"id\":\"pu_output\",\"label\":\"o\",\"type\":\"output\"}],\"Top\":[]}"
  Simulink-PS Converter : nesl_utility/Simulink-PS Converter  PhysicalDomain=network_engine_domain  SubClassName=ps_input  LeftPortType=input  RightPortType=output  PseudoPeriodic=off  Frequencies=[]  NoiseDistribution=none  NoiseParameters=[]  Unit=1  AffineConversion=off  FilteringAndDerivatives=provide  SimscapeFilterOrder=1  InputFilterTimeConstant=0.001  UdotUserProvided=0
  Unit Delay : UnitDelay  InitialCondition=1  SampleTime=Ts  HasFrameUpgradeWarning=on
  wref : Constant
  R : PMIOPort  Side=Right
  C : PMIOPort  Port=2  Side=Right
  pu : PMIOPort  Port=3  Side=Left
  wires:
  PS-Simulink Converter/1 -> Unit Delay/1
  Unit Delay/1 -> "Governor and Prime Mover "/3(w)
  Pref/1 -> "Governor and Prime Mover "/2(Pref)
  "Governor and Prime Mover "/1(Tm) -> Simulink-PS Converter/1
  wref/1 -> "Governor and Prime Mover "/1(wref)
  connections:
  PS-Simulink Converter/LConn1 -- Rotor velocity measurement/RConn1
  Mechanical Power/RConn1 -- R/RConn1
  pu/RConn1 -- Rotor velocity measurement/LConn1
  Mechanical Power/RConn2 -- C/RConn1
  Mechanical Power/LConn1 -- Simulink-PS Converter/RConn1

== system IEEE9BusSystem/Gen1@Bus1 Swing/Governor and Prime Mover/Governor and Prime Mover  ==
  wref : Inport
  Pref : Inport  Port=2
  w : Inport  Port=3
  Governor : Subsystem
  Non-reheat turbine : Subsystem
  Tm : Outport  VectorParamsAs1DForOutWhenUnconnected=off
  wires:
  w/1 -> Governor/3(w)
  Pref/1 -> Governor/2(Pref)
  wref/1 -> Governor/1(wref)
  Non-reheat turbine/1(torque) -> Tm/1
  Governor/1(delta_y) -> Non-reheat turbine/1(delta_y)

== system IEEE9BusSystem/Gen2@Bus2 PV 1.025 pu 163 MW/Governor and Prime Mover/Governor and Prime Mover  ==
  wref : Inport
  Pref : Inport  Port=2
  w : Inport  Port=3
  Governor : Subsystem
  Non-reheat turbine : Subsystem
  Tm : Outport  VectorParamsAs1DForOutWhenUnconnected=off
  wires:
  Governor/1(delta_y) -> Non-reheat turbine/1(delta_y)
  Non-reheat turbine/1(torque) -> Tm/1
  wref/1 -> Governor/1(wref)
  Pref/1 -> Governor/2(Pref)
  w/1 -> Governor/3(w)

== system IEEE9BusSystem/Gen3@Bus3 PV 1.025 pu 85 MW/Governor and Prime Mover/Governor and Prime Mover  ==
  wref : Inport
  Pref : Inport  Port=2
  w : Inport  Port=3
  Governor : Subsystem
  Non-reheat turbine : Subsystem
  Tm : Outport  VectorParamsAs1DForOutWhenUnconnected=off
  wires:
  w/1 -> Governor/3(w)
  Pref/1 -> Governor/2(Pref)
  wref/1 -> Governor/1(wref)
  Non-reheat turbine/1(torque) -> Tm/1
  Governor/1(delta_y) -> Non-reheat turbine/1(delta_y)

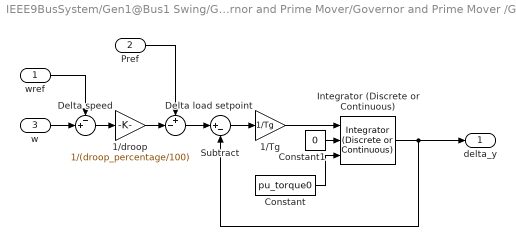
== system IEEE9BusSystem/Gen1@Bus1 Swing/Governor and Prime Mover/Governor and Prime Mover /Governor ==
  wref : Inport
  Pref : Inport  Port=2
  w : Inport  Port=3
  1/Tg : Gain  Gain=1/Tg
  1/droop : Gain  Gain=1/(droop_percentage/100)
  Constant : Constant  Value=pu_torque0
  Constant1 : Constant  Value=0
  Delta load setpoint : Sum  Inputs=+-|
  Delta speed : Sum  Inputs=-+|
  Integrator (Discrete or Continuous) : eeGeneralControl/Integrator (Discrete or Continuous)  LabelModeActiveChoice=Discrete  ExternalReset=level  LimitType=Anti-windup  B=inf  A=-inf  Ts=Ts
  Subtract : Sum  Inputs=|+-
  delta_y : Outport  VectorParamsAs1DForOutWhenUnconnected=off
  wires:
  Constant1/1 -> Integrator (Discrete or Continuous)/2
  Constant/1 -> Integrator (Discrete or Continuous)/3
  Pref/1 -> Delta load setpoint/1
  wref/1 -> Delta speed/1
  Integrator (Discrete or Continuous)/1 -> Subtract/2, delta_y/1
  1/Tg/1 -> Integrator (Discrete or Continuous)/1
  Subtract/1 -> 1/Tg/1
  Delta load setpoint/1 -> Subtract/1
  1/droop/1 -> Delta load setpoint/2
  w/1 -> Delta speed/2
  Delta speed/1 -> 1/droop/1

== system IEEE9BusSystem/Gen1@Bus1 Swing/Governor and Prime Mover/Governor and Prime Mover /Non-reheat turbine ==
  delta_y : Inport
  1/Tch : Gain  Gain=1/Tch
  Constant : Constant  Value=pu_torque0
  Constant1 : Constant  Value=0
  Integrator (Discrete or Continuous) : eeGeneralControl/Integrator (Discrete or Continuous)  LabelModeActiveChoice=Discrete  ExternalReset=level  LimitType=Anti-windup  B=inf  A=-inf  Ts=Ts
  Sum : Sum  Inputs=|+-
  torque : Outport  VectorParamsAs1DForOutWhenUnconnected=off
  wires:
  Constant/1 -> Integrator (Discrete or Continuous)/3
  Constant1/1 -> Integrator (Discrete or Continuous)/2
  Integrator (Discrete or Continuous)/1 -> torque/1, Sum/2
  1/Tch/1 -> Integrator (Discrete or Continuous)/1
  Sum/1 -> 1/Tch/1
  delta_y/1 -> Sum/1

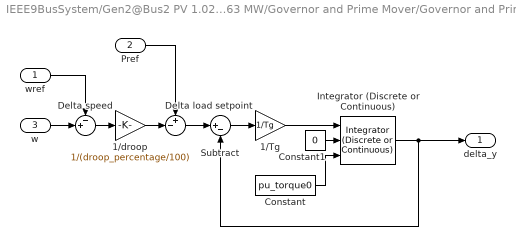
== system IEEE9BusSystem/Gen2@Bus2 PV 1.025 pu 163 MW/Governor and Prime Mover/Governor and Prime Mover /Governor ==
  wref : Inport
  Pref : Inport  Port=2
  w : Inport  Port=3
  1/Tg : Gain  Gain=1/Tg
  1/droop : Gain  Gain=1/(droop_percentage/100)
  Constant : Constant  Value=pu_torque0
  Constant1 : Constant  Value=0
  Delta load setpoint : Sum  Inputs=+-|
  Delta speed : Sum  Inputs=-+|
  Integrator (Discrete or Continuous) : eeGeneralControl/Integrator (Discrete or Continuous)  LabelModeActiveChoice=Discrete  ExternalReset=level  LimitType=Anti-windup  B=inf  A=-inf  Ts=Ts
  Subtract : Sum  Inputs=|+-
  delta_y : Outport  VectorParamsAs1DForOutWhenUnconnected=off
  wires:
  Delta speed/1 -> 1/droop/1
  w/1 -> Delta speed/2
  1/droop/1 -> Delta load setpoint/2
  Delta load setpoint/1 -> Subtract/1
  Subtract/1 -> 1/Tg/1
  1/Tg/1 -> Integrator (Discrete or Continuous)/1
  Integrator (Discrete or Continuous)/1 -> delta_y/1, Subtract/2
  wref/1 -> Delta speed/1
  Pref/1 -> Delta load setpoint/1
  Constant/1 -> Integrator (Discrete or Continuous)/3
  Constant1/1 -> Integrator (Discrete or Continuous)/2

== system IEEE9BusSystem/Gen2@Bus2 PV 1.025 pu 163 MW/Governor and Prime Mover/Governor and Prime Mover /Non-reheat turbine ==
  delta_y : Inport
  1/Tch : Gain  Gain=1/Tch
  Constant : Constant  Value=pu_torque0
  Constant1 : Constant  Value=0
  Integrator (Discrete or Continuous) : eeGeneralControl/Integrator (Discrete or Continuous)  LabelModeActiveChoice=Discrete  ExternalReset=level  LimitType=Anti-windup  B=inf  A=-inf  Ts=Ts
  Sum : Sum  Inputs=|+-
  torque : Outport  VectorParamsAs1DForOutWhenUnconnected=off
  wires:
  delta_y/1 -> Sum/1
  Sum/1 -> 1/Tch/1
  1/Tch/1 -> Integrator (Discrete or Continuous)/1
  Integrator (Discrete or Continuous)/1 -> Sum/2, torque/1
  Constant1/1 -> Integrator (Discrete or Continuous)/2
  Constant/1 -> Integrator (Discrete or Continuous)/3

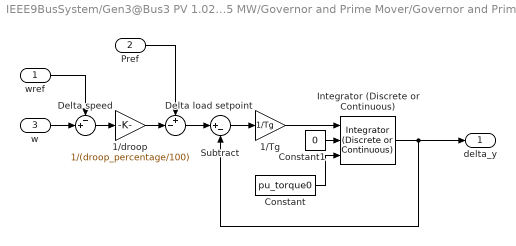
== system IEEE9BusSystem/Gen3@Bus3 PV 1.025 pu 85 MW/Governor and Prime Mover/Governor and Prime Mover /Governor ==
  wref : Inport
  Pref : Inport  Port=2
  w : Inport  Port=3
  1/Tg : Gain  Gain=1/Tg
  1/droop : Gain  Gain=1/(droop_percentage/100)
  Constant : Constant  Value=pu_torque0
  Constant1 : Constant  Value=0
  Delta load setpoint : Sum  Inputs=+-|
  Delta speed : Sum  Inputs=-+|
  Integrator (Discrete or Continuous) : eeGeneralControl/Integrator (Discrete or Continuous)  LabelModeActiveChoice=Discrete  ExternalReset=level  LimitType=Anti-windup  B=inf  A=-inf  Ts=Ts
  Subtract : Sum  Inputs=|+-
  delta_y : Outport  VectorParamsAs1DForOutWhenUnconnected=off
  wires:
  Constant1/1 -> Integrator (Discrete or Continuous)/2
  Constant/1 -> Integrator (Discrete or Continuous)/3
  Pref/1 -> Delta load setpoint/1
  wref/1 -> Delta speed/1
  Integrator (Discrete or Continuous)/1 -> Subtract/2, delta_y/1
  1/Tg/1 -> Integrator (Discrete or Continuous)/1
  Subtract/1 -> 1/Tg/1
  Delta load setpoint/1 -> Subtract/1
  1/droop/1 -> Delta load setpoint/2
  w/1 -> Delta speed/2
  Delta speed/1 -> 1/droop/1

== system IEEE9BusSystem/Gen3@Bus3 PV 1.025 pu 85 MW/Governor and Prime Mover/Governor and Prime Mover /Non-reheat turbine ==
  delta_y : Inport
  1/Tch : Gain  Gain=1/Tch
  Constant : Constant  Value=pu_torque0
  Constant1 : Constant  Value=0
  Integrator (Discrete or Continuous) : eeGeneralControl/Integrator (Discrete or Continuous)  LabelModeActiveChoice=Discrete  ExternalReset=level  LimitType=Anti-windup  B=inf  A=-inf  Ts=Ts
  Sum : Sum  Inputs=|+-
  torque : Outport  VectorParamsAs1DForOutWhenUnconnected=off
  wires:
  Constant/1 -> Integrator (Discrete or Continuous)/3
  Constant1/1 -> Integrator (Discrete or Continuous)/2
  Integrator (Discrete or Continuous)/1 -> torque/1, Sum/2
  1/Tch/1 -> Integrator (Discrete or Continuous)/1
  Sum/1 -> 1/Tch/1
  delta_y/1 -> Sum/1
